simulink model "HarnessModel_MotorDriveUnit"  (R2026a)
settings: Solver=daessc  StopTime=10
PreLoadFcn:
  | MDU_HarnessInputs.AxleSpeedSwitch = table( ...
  |   simscape.Value([0 1], "s"), ...
  |   [0 0], ...
  |   VariableNames=["Time" "StepValues"]);
  | 
  | MDU_HarnessInputs.AxleSpeed = table( ...
  |   simscape.Value([0 1 2], "s"), ...
  |   simscape.Value([0 0 0], "rpm"), ...
  |   VariableNames=["Time" "Data"]);
  | 
  | MDU_HarnessInputs.AxleTorque = table( ...
  |   simscape.Value([0 1 2], "s"), ...
  |   simscape.Value([0 0 0], "N*m"), ...
  |   VariableNames=["Time" "Data"]);
  | 
  | MDU_HarnessInputs.MotorTorqueCommand = table( ...
  |   simscape.Value([0 1 2], "s"), ...
  |   simscape.Value([0 0 0], "N*m"), ...
  |   VariableNames=["Time" "Data"]);
  | 
  | MDU_HarnessInputs.MotorHeatFlow = table( ...
  |   simscape.Value([0 1 2], "s"), ...
  |   simscape.Value([0 0 0], "W"), ...
  |   VariableNames=["Time" "Data"]);
  | 
  | setupHarness_MotorDriveUnit
undefined symbols (not defined in the file or in its folder): BatteryHV, initial, MechanicalLoad, Minus, Plus
libraries: fl_lib x22, nesl_utility x10, sdl_lib x1
settings Model: Creator=isaacito  LastModifiedBy=ythvg
settings SimscapeCC: SimscapeNominalValues="[{\"value\":\"1\",\"unit\":\"A\"},{\"value\":\"1\",\"unit\":\"bar\"},{\"value\":\"1\",\"unit\":\"cm^2\"},{\"value\":\"1\",\"unit\":\"cm^3/s\"},{\"value\":\"1\",\"unit\":\"kJ/kg\"},{\"value\":\"1\",\"unit\":\"kW\"},{\"value\":\"1\",\"unit\":\"l\"},{\"value\":\"1\",\"unit\":\"N\"},{\"value\":\"1\",\"unit\":\"N*m\"},{\"value\":\"1\",\"unit\":\"V\"}]"  SimscapeLogSimulationStatistics=on  SimscapeLogLimitData=off  SimscapeLogDataHistory=5000.0

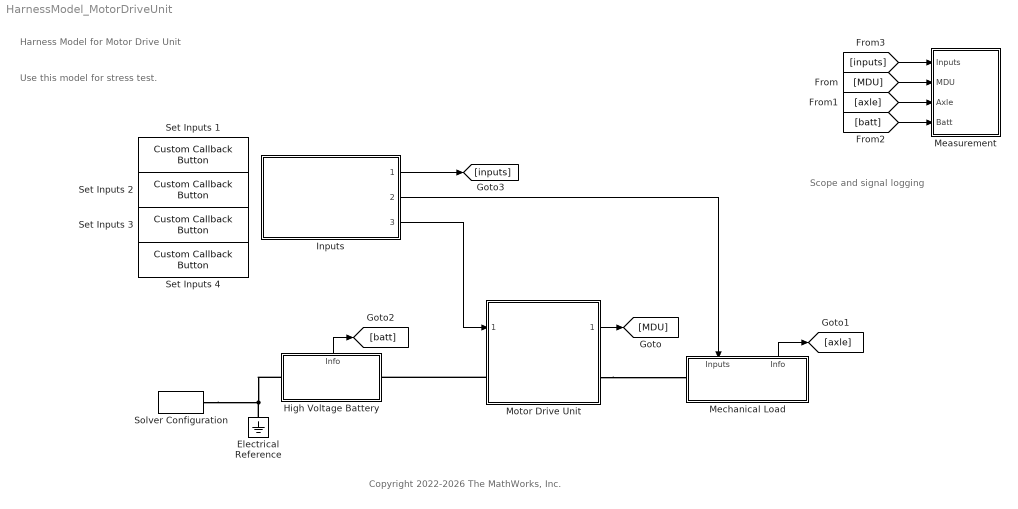
== system HarnessModel_MotorDriveUnit ==
  note: Harness Model for Motor Drive Unit
  note: Copyright 2022-2026 The MathWorks, Inc.
  note: Use this model for stress test.
  note: Scope and signal logging
  Electrical Reference : fl_lib/Electrical/Electrical Elements/Electrical Reference
  High Voltage Battery : Subsystem
      settings: PortSchema="{\"entries\":[{\"content\":{\"sides\":[{\"content\":{\"connectorIds\":[\"LConn1\"]},\"type\":\"ConnectorPlacement.EquallySpacedRectSide\",\"uuid\":\"8acd7e9a-bb08-4de6-aa14-0989ebba81b9\"},{\"content\":{\"connectorIds\":[\"RConn1\"],\"side\":\"RIGHT\"},\"type\":\"ConnectorPlacement.EquallySpacedRectSide\",\"uuid\":\"f80e1afc-966f-4d6b-84f9-f0b60dd6f20c\"},{\"content\":{\"connectorIds\":[\"Out1\"],\"side\":\"TOP\"},\"type\":\"ConnectorPlacement.EquallySpacedRectSide\",\"uuid\":\"52ccb2b1-bd5e-4dcb-b9b6-0ef03b912c33\"}]},\"type\":\"ConnectorPlacement.EquallySpacedConnector\",\"uuid\":\"b55f48a4-f283-4a77-8513-99b31abb285a\"}],\"packageUris\":[\"http://schema.mathworks.com/mf0/Connector/R2020b\"],\"version\":\"1.0\"}"
  Inputs : Subsystem  ReferencedSubsystem=Inputs_MotorDriveUnit_LookupTable_refsub
      settings: OpenFcn="open_system(gcb, \"force\")"
  Measurement : Subsystem
  Mechanical Load : Subsystem
      settings: PortSchema="{\"entries\":[{\"content\":{\"sides\":[{\"content\":{\"connectorIds\":[\"LConn1\"]},\"type\":\"ConnectorPlacement.EquallySpacedRectSide\",\"uuid\":\"18221845-08ef-4cf2-b090-320221152030\"},{\"content\":{\"connectorIds\":[],\"side\":\"RIGHT\"},\"type\":\"ConnectorPlacement.EquallySpacedRectSide\",\"uuid\":\"d5b0548b-74c8-455a-9783-7dc299f3571f\"},{\"content\":{\"connectorIds\":[\"In1\",\"Out1\"],\"side\":\"TOP\"},\"type\":\"ConnectorPlacement.EquallySpacedRectSide\",\"uuid\":\"542d8e55-6d7f-4c9a-9fdc-66897ed9f466\"}]},\"type\":\"ConnectorPlacement.EquallySpacedConnector\",\"uuid\":\"3cd4c536-0337-4305-a842-969bfb1fefe3\"}],\"packageUris\":[\"http://schema.mathworks.com/mf0/Connector/R2020b\"],\"version\":\"1.0\"}"
  Motor Drive Unit : Subsystem  ReferencedSubsystem=MotorDriveUnit_Basic_refsub
      settings: OpenFcn=|
      | % Look under mask:
      | open_system(gcb, "force")
  Set Inputs 1 : CustomCallbackButton  Configuration="{\"components\":[{\"name\":\"BackgroundImageComponent\",\"settings\":{\"image\":{\"size\":[0,0],\"src\":\"default\",\"srcOrientation\":\"Right\"},\"position\":[0,0,1,1]}},{\"name\":\"ButtonStateComponent\",\"settings\":{\"buttonType\":\"momentary\",\"clickFcn\":\"disp(\\\"Loading inputs: <a href=\\\"\\\"matlab:edit('LoadInputs_MotorDriveUnit_zero')\\\"\\\">LoadInputs_MotorDriveUnit_zero<\\/a>\\\")\\nLoadInputs_MotorDriveUnit_zero\\n\\nset_param(bdroot, StopTime=\\\"10\\\")\\nset_param(gcs + \\\"\\/Inputs\\\", ReferencedSubsystem = \\\"Inputs_MotorDriveUnit_LookupTable_refsub\\\")\\n\",\"onValue\":1,\"position\":[0,0,1,1],\"pressDelay\":\"500\",\"pressFcn\":\"\",\"repeatInterval\":\"0\",\"states\":[{\"horizontalAlignment\":\"center\",\"image\":{\"position\":[0,0,1,1],\"size\":[1,1],\"src\":\"default\",\"srcOrientation\":\"Right\"},\"label\":{\"color\":[0.01176470588,0.01176470588,0.01176470588,1],\"icon\":{\"size\":[0,0],\"src\":\"default\",\"srcOrientation\":\"Right\"},\"iconOffset\":0,\"iconPlacement\":\"left\",\"opacity\":1,\"show\":true,\"text\":{\"content\":\"Constant\",\"font\":\"Helvetica\"}},\"labelOffset\":[0,0],\"verticalAlignment\":\"middle\"},{\"horizontalAlignment\":\"center\",\"image\":{\"position\":[0,0,1,1],\"size\":[1,1],\"src\":\"default\",\"srcOrientation\":\"Right\"},\"label\":{\"color\":[0.01176470588,0.01176470588,0.01176470588,1],\"icon\":{\"size\":[0,0],\"src\":\"default\",\"srcOrientation\":\"Right\"},\"iconOffset\":0,\"iconPlacement\":\"left\",\"opacity\":1,\"show\":true,\"text\":{\"content\":\"Constant\",\"font\":\"Helvetica\"}},\"labelOffset\":[0,0],\"verticalAlignment\":\"middle\"},{\"horizontalAlignment\":\"center\",\"image\":{\"position\":[0,0,1,1],\"size\":[1,1],\"src\":\"default\",\"srcOrientation\":\"Right\"},\"label\":{\"color\":[0.01176470588,0.01176470588,0.01176470588,1],\"icon\":{\"size\":[0,0],\"src\":\"default\",\"srcOrientation\":\"Right\"},\"iconOffset\":0,\"iconPlacement\":\"left\",\"opacity\":1,\"show\":true,\"text\":{\"content\":\"Constant\",\"font\":\"Helvetica\"}},\"labelOffset\":[0,0],\"verticalAlignment\":\"middle\"},{\"horizontalAlignment\":\"center\",\"image\":{\"position\":[0,0,1,1],\"size\":[1,1],\"src\":\"default\",\"srcOrientation\":\"Right\"},\"label\":{\"color\":[0.01176470588,0.01176470588,0.01176470588,1],\"icon\":{\"size\":[0,0],\"src\":\"default\",\"srcOrientation\":\"Right\"},\"iconOffset\":0,\"iconPlacement\":\"left\",\"opacity\":1,\"show\":true,\"text\":{\"content\":\"Constant\",\"font\":\"Helvetica\"}},\"labelOffset\":[0,0],\"verticalAlignment\":\"middle\"}]}},{\"name\":\"ForegroundImageComponent\",\"settings\":{\"image\":{\"size\":[0,0],\"src\":\"default\",\"srcOrientation\":\"Right\"},\"isForeground\":1,\"position\":[0,0,1,1]}}],\"derived\":{\"blockParameters\":{\"AutoActivate\":true,\"ButtonText\":\"Constant\",\"ButtonType\":\"Momentary\",\"ClickFcn\":\"disp(\\\"Loading inputs: <a href=\\\"\\\"matlab:edit('LoadInputs_MotorDriveUnit_zero')\\\"\\\">LoadInputs_MotorDriveUnit_zero<\\/a>\\\")\\nLoadInputs_MotorDriveUnit_zero\\n\\nset_param(bdroot, StopTime=\\\"10\\\")\\nset_param(gcs + \\\"\\/Inputs\\\", ReferencedSubsystem = \\\"Inputs_MotorDriveUnit_LookupTable_refsub\\\")\\n\",\"OnValue\":1,\"PressDelay\":\"500\",\"PressFcn\":\"\",\"RepeatInterval\":\"0\",\"fixedAspectRatio\":\"on\"}},\"settings\":{\"BindingType\":\"standalone\",\"autoActivate\":true,\"backgroundColor\":[244,244,244,1],\"backgroundOffset\":0.2,\"backgroundOpacity\":1,\"fixedAspectRatio\":\"on\",\"foregroundColor\":[0.01176470588,0.01176470588,0.01176470588,1],\"migratedFromLegacy\":true,\"useBackgroundColor\":true,\"variant\":\"callback\",\"version\":\"R2025a\"},\"type\":\"Button\"}"  CustomBackgroundColor="{\"color\":[0.9568627451,0.9568627451,0.9568627451],\"show\":true}"
  Set Inputs 2 : CustomCallbackButton  Configuration="{\"components\":[{\"name\":\"BackgroundImageComponent\",\"settings\":{\"image\":{\"size\":[0,0],\"src\":\"default\",\"srcOrientation\":\"Right\"},\"position\":[0,0,1,1]}},{\"name\":\"ButtonStateComponent\",\"settings\":{\"buttonType\":\"momentary\",\"clickFcn\":\"disp(\\\"Loading inputs: <a href=\\\"\\\"matlab:edit('LoadInputs_MotorDriveUnit_Drive')\\\"\\\">LoadInputs_MotorDriveUnit_Drive<\\/a>\\\")\\nLoadInputs_MotorDriveUnit_Drive\\n\\nset_param(bdroot, StopTime=\\\"300\\\")\\nset_param(gcs + \\\"\\/Inputs\\\", ReferencedSubsystem = \\\"Inputs_MotorDriveUnit_LookupTable_refsub\\\")\\n\",\"onValue\":1,\"position\":[0,0,1,1],\"pressDelay\":\"500\",\"pressFcn\":\"\",\"repeatInterval\":\"0\",\"states\":[{\"horizontalAlignment\":\"center\",\"image\":{\"position\":[0,0,1,1],\"size\":[1,1],\"src\":\"default\",\"srcOrientation\":\"Right\"},\"label\":{\"color\":[0.01176470588,0.01176470588,0.01176470588,1],\"icon\":{\"size\":[0,0],\"src\":\"default\",\"srcOrientation\":\"Right\"},\"iconOffset\":0,\"iconPlacement\":\"left\",\"opacity\":1,\"show\":true,\"text\":{\"content\":\"Drive\",\"font\":\"Helvetica\"}},\"labelOffset\":[0,0],\"verticalAlignment\":\"middle\"},{\"horizontalAlignment\":\"center\",\"image\":{\"position\":[0,0,1,1],\"size\":[1,1],\"src\":\"default\",\"srcOrientation\":\"Right\"},\"label\":{\"color\":[0.01176470588,0.01176470588,0.01176470588,1],\"icon\":{\"size\":[0,0],\"src\":\"default\",\"srcOrientation\":\"Right\"},\"iconOffset\":0,\"iconPlacement\":\"left\",\"opacity\":1,\"show\":true,\"text\":{\"content\":\"Drive\",\"font\":\"Helvetica\"}},\"labelOffset\":[0,0],\"verticalAlignment\":\"middle\"},{\"horizontalAlignment\":\"center\",\"image\":{\"position\":[0,0,1,1],\"size\":[1,1],\"src\":\"default\",\"srcOrientation\":\"Right\"},\"label\":{\"color\":[0.01176470588,0.01176470588,0.01176470588,1],\"icon\":{\"size\":[0,0],\"src\":\"default\",\"srcOrientation\":\"Right\"},\"iconOffset\":0,\"iconPlacement\":\"left\",\"opacity\":1,\"show\":true,\"text\":{\"content\":\"Drive\",\"font\":\"Helvetica\"}},\"labelOffset\":[0,0],\"verticalAlignment\":\"middle\"},{\"horizontalAlignment\":\"center\",\"image\":{\"position\":[0,0,1,1],\"size\":[1,1],\"src\":\"default\",\"srcOrientation\":\"Right\"},\"label\":{\"color\":[0.01176470588,0.01176470588,0.01176470588,1],\"icon\":{\"size\":[0,0],\"src\":\"default\",\"srcOrientation\":\"Right\"},\"iconOffset\":0,\"iconPlacement\":\"left\",\"opacity\":1,\"show\":true,\"text\":{\"content\":\"Drive\",\"font\":\"Helvetica\"}},\"labelOffset\":[0,0],\"verticalAlignment\":\"middle\"}]}},{\"name\":\"ForegroundImageComponent\",\"settings\":{\"image\":{\"size\":[0,0],\"src\":\"default\",\"srcOrientation\":\"Right\"},\"isForeground\":1,\"position\":[0,0,1,1]}}],\"derived\":{\"blockParameters\":{\"AutoActivate\":true,\"ButtonText\":\"Drive\",\"ButtonType\":\"Momentary\",\"ClickFcn\":\"disp(\\\"Loading inputs: <a href=\\\"\\\"matlab:edit('LoadInputs_MotorDriveUnit_Drive')\\\"\\\">LoadInputs_MotorDriveUnit_Drive<\\/a>\\\")\\nLoadInputs_MotorDriveUnit_Drive\\n\\nset_param(bdroot, StopTime=\\\"300\\\")\\nset_param(gcs + \\\"\\/Inputs\\\", ReferencedSubsystem = \\\"Inputs_MotorDriveUnit_LookupTable_refsub\\\")\\n\",\"OnValue\":1,\"PressDelay\":\"500\",\"PressFcn\":\"\",\"RepeatInterval\":\"0\",\"fixedAspectRatio\":\"on\"}},\"settings\":{\"BindingType\":\"standalone\",\"autoActivate\":true,\"backgroundColor\":[244,244,244,1],\"backgroundOffset\":0.2,\"backgroundOpacity\":1,\"fixedAspectRatio\":\"on\",\"foregroundColor\":[0.01176470588,0.01176470588,0.01176470588,1],\"migratedFromLegacy\":true,\"useBackgroundColor\":true,\"variant\":\"callback\",\"version\":\"R2025a\"},\"type\":\"Button\"}"  CustomBackgroundColor="{\"color\":[0.9568627451,0.9568627451,0.9568627451],\"show\":true}"
  Set Inputs 3 : CustomCallbackButton  Configuration="{\"components\":[{\"name\":\"BackgroundImageComponent\",\"settings\":{\"image\":{\"size\":[0,0],\"src\":\"default\",\"srcOrientation\":\"Right\"},\"position\":[0,0,1,1]}},{\"name\":\"ButtonStateComponent\",\"settings\":{\"buttonType\":\"momentary\",\"clickFcn\":\"disp(\\\"Loading inputs: <a href=\\\"\\\"matlab:edit('LoadInputs_MotorDriveUnit_Regen')\\\"\\\">LoadInputs_MotorDriveUnit_Regen<\\/a>\\\")\\nLoadInputs_MotorDriveUnit_Regen\\n\\nset_param(bdroot, StopTime=\\\"400\\\")\\nset_param(gcs + \\\"\\/Inputs\\\", ReferencedSubsystem = \\\"Inputs_MotorDriveUnit_LookupTable_refsub\\\")\\n\",\"onValue\":1,\"position\":[0,0,1,1],\"pressDelay\":\"500\",\"pressFcn\":\"\",\"repeatInterval\":\"0\",\"states\":[{\"horizontalAlignment\":\"center\",\"image\":{\"position\":[0,0,1,1],\"size\":[1,1],\"src\":\"default\",\"srcOrientation\":\"Right\"},\"label\":{\"color\":[0.01176470588,0.01176470588,0.01176470588,1],\"icon\":{\"size\":[0,0],\"src\":\"default\",\"srcOrientation\":\"Right\"},\"iconOffset\":0,\"iconPlacement\":\"left\",\"opacity\":1,\"show\":true,\"text\":{\"content\":\"Regen Brake\",\"font\":\"Helvetica\"}},\"labelOffset\":[0,0],\"verticalAlignment\":\"middle\"},{\"horizontalAlignment\":\"center\",\"image\":{\"position\":[0,0,1,1],\"size\":[1,1],\"src\":\"default\",\"srcOrientation\":\"Right\"},\"label\":{\"color\":[0.01176470588,0.01176470588,0.01176470588,1],\"icon\":{\"size\":[0,0],\"src\":\"default\",\"srcOrientation\":\"Right\"},\"iconOffset\":0,\"iconPlacement\":\"left\",\"opacity\":1,\"show\":true,\"text\":{\"content\":\"Regen Brake\",\"font\":\"Helvetica\"}},\"labelOffset\":[0,0],\"verticalAlignment\":\"middle\"},{\"horizontalAlignment\":\"center\",\"image\":{\"position\":[0,0,1,1],\"size\":[1,1],\"src\":\"default\",\"srcOrientation\":\"Right\"},\"label\":{\"color\":[0.01176470588,0.01176470588,0.01176470588,1],\"icon\":{\"size\":[0,0],\"src\":\"default\",\"srcOrientation\":\"Right\"},\"iconOffset\":0,\"iconPlacement\":\"left\",\"opacity\":1,\"show\":true,\"text\":{\"content\":\"Regen Brake\",\"font\":\"Helvetica\"}},\"labelOffset\":[0,0],\"verticalAlignment\":\"middle\"},{\"horizontalAlignment\":\"center\",\"image\":{\"position\":[0,0,1,1],\"size\":[1,1],\"src\":\"default\",\"srcOrientation\":\"Right\"},\"label\":{\"color\":[0.01176470588,0.01176470588,0.01176470588,1],\"icon\":{\"size\":[0,0],\"src\":\"default\",\"srcOrientation\":\"Right\"},\"iconOffset\":0,\"iconPlacement\":\"left\",\"opacity\":1,\"show\":true,\"text\":{\"content\":\"Regen Brake\",\"font\":\"Helvetica\"}},\"labelOffset\":[0,0],\"verticalAlignment\":\"middle\"}]}},{\"name\":\"ForegroundImageComponent\",\"settings\":{\"image\":{\"size\":[0,0],\"src\":\"default\",\"srcOrientation\":\"Right\"},\"isForeground\":1,\"position\":[0,0,1,1]}}],\"derived\":{\"blockParameters\":{\"AutoActivate\":true,\"ButtonText\":\"Regen Brake\",\"ButtonType\":\"Momentary\",\"ClickFcn\":\"disp(\\\"Loading inputs: <a href=\\\"\\\"matlab:edit('LoadInputs_MotorDriveUnit_Regen')\\\"\\\">LoadInputs_MotorDriveUnit_Regen<\\/a>\\\")\\nLoadInputs_MotorDriveUnit_Regen\\n\\nset_param(bdroot, StopTime=\\\"400\\\")\\nset_param(gcs + \\\"\\/Inputs\\\", ReferencedSubsystem = \\\"Inputs_MotorDriveUnit_LookupTable_refsub\\\")\\n\",\"OnValue\":1,\"PressDelay\":\"500\",\"PressFcn\":\"\",\"RepeatInterval\":\"0\",\"fixedAspectRatio\":\"on\"}},\"settings\":{\"BindingType\":\"standalone\",\"autoActivate\":true,\"backgroundColor\":[244,244,244,1],\"backgroundOffset\":0.2,\"backgroundOpacity\":1,\"fixedAspectRatio\":\"on\",\"foregroundColor\":[0.01176470588,0.01176470588,0.01176470588,1],\"migratedFromLegacy\":true,\"useBackgroundColor\":true,\"variant\":\"callback\",\"version\":\"R2025a\"},\"type\":\"Button\"}"  CustomBackgroundColor="{\"color\":[0.9568627451,0.9568627451,0.9568627451],\"show\":true}"
  Set Inputs 4 : CustomCallbackButton  Configuration="{\"components\":[{\"name\":\"BackgroundImageComponent\",\"settings\":{\"image\":{\"size\":[0,0],\"src\":\"default\",\"srcOrientation\":\"Right\"},\"position\":[0,0,1,1]}},{\"name\":\"ButtonStateComponent\",\"settings\":{\"buttonType\":\"momentary\",\"clickFcn\":\"disp(\\\"Loading inputs: <a href=\\\"\\\"matlab:edit('LoadInputs_MotorDriveUnit_Random')\\\"\\\">LoadInputs_MotorDriveUnit_Random<\\/a>\\\")\\nLoadInputs_MotorDriveUnit_Random\\n\\nset_param(bdroot, StopTime=\\\"400\\\")\\nset_param(gcs + \\\"\\/Inputs\\\", ReferencedSubsystem = \\\"Inputs_MotorDriveUnit_LookupTable_refsub\\\")\\n\",\"onValue\":1,\"position\":[0,0,1,1],\"pressDelay\":\"500\",\"pressFcn\":\"\",\"repeatInterval\":\"0\",\"states\":[{\"horizontalAlignment\":\"center\",\"image\":{\"position\":[0,0,1,1],\"size\":[1,1],\"src\":\"default\",\"srcOrientation\":\"Right\"},\"label\":{\"color\":[0.01176470588,0.01176470588,0.01176470588,1],\"icon\":{\"size\":[0,0],\"src\":\"default\",\"srcOrientation\":\"Right\"},\"iconOffset\":0,\"iconPlacement\":\"left\",\"opacity\":1,\"show\":true,\"text\":{\"content\":\"Random\",\"font\":\"Helvetica\"}},\"labelOffset\":[0,0],\"verticalAlignment\":\"middle\"},{\"horizontalAlignment\":\"center\",\"image\":{\"position\":[0,0,1,1],\"size\":[1,1],\"src\":\"default\",\"srcOrientation\":\"Right\"},\"label\":{\"color\":[0.01176470588,0.01176470588,0.01176470588,1],\"icon\":{\"size\":[0,0],\"src\":\"default\",\"srcOrientation\":\"Right\"},\"iconOffset\":0,\"iconPlacement\":\"left\",\"opacity\":1,\"show\":true,\"text\":{\"content\":\"Random\",\"font\":\"Helvetica\"}},\"labelOffset\":[0,0],\"verticalAlignment\":\"middle\"},{\"horizontalAlignment\":\"center\",\"image\":{\"position\":[0,0,1,1],\"size\":[1,1],\"src\":\"default\",\"srcOrientation\":\"Right\"},\"label\":{\"color\":[0.01176470588,0.01176470588,0.01176470588,1],\"icon\":{\"size\":[0,0],\"src\":\"default\",\"srcOrientation\":\"Right\"},\"iconOffset\":0,\"iconPlacement\":\"left\",\"opacity\":1,\"show\":true,\"text\":{\"content\":\"Random\",\"font\":\"Helvetica\"}},\"labelOffset\":[0,0],\"verticalAlignment\":\"middle\"},{\"horizontalAlignment\":\"center\",\"image\":{\"position\":[0,0,1,1],\"size\":[1,1],\"src\":\"default\",\"srcOrientation\":\"Right\"},\"label\":{\"color\":[0.01176470588,0.01176470588,0.01176470588,1],\"icon\":{\"size\":[0,0],\"src\":\"default\",\"srcOrientation\":\"Right\"},\"iconOffset\":0,\"iconPlacement\":\"left\",\"opacity\":1,\"show\":true,\"text\":{\"content\":\"Random\",\"font\":\"Helvetica\"}},\"labelOffset\":[0,0],\"verticalAlignment\":\"middle\"}]}},{\"name\":\"ForegroundImageComponent\",\"settings\":{\"image\":{\"size\":[0,0],\"src\":\"default\",\"srcOrientation\":\"Right\"},\"isForeground\":1,\"position\":[0,0,1,1]}}],\"derived\":{\"blockParameters\":{\"AutoActivate\":true,\"ButtonText\":\"Random\",\"ButtonType\":\"Momentary\",\"ClickFcn\":\"disp(\\\"Loading inputs: <a href=\\\"\\\"matlab:edit('LoadInputs_MotorDriveUnit_Random')\\\"\\\">LoadInputs_MotorDriveUnit_Random<\\/a>\\\")\\nLoadInputs_MotorDriveUnit_Random\\n\\nset_param(bdroot, StopTime=\\\"400\\\")\\nset_param(gcs + \\\"\\/Inputs\\\", ReferencedSubsystem = \\\"Inputs_MotorDriveUnit_LookupTable_refsub\\\")\\n\",\"OnValue\":1,\"PressDelay\":\"500\",\"PressFcn\":\"\",\"RepeatInterval\":\"0\",\"fixedAspectRatio\":\"on\"}},\"settings\":{\"BindingType\":\"standalone\",\"autoActivate\":true,\"backgroundColor\":[244,244,244,1],\"backgroundOffset\":0.2,\"backgroundOpacity\":1,\"fixedAspectRatio\":\"on\",\"foregroundColor\":[0.01176470588,0.01176470588,0.01176470588,1],\"migratedFromLegacy\":true,\"useBackgroundColor\":true,\"variant\":\"callback\",\"version\":\"R2025a\"},\"type\":\"Button\"}"  CustomBackgroundColor="{\"color\":[0.9568627451,0.9568627451,0.9568627451],\"show\":true}"
  Solver Configuration : nesl_utility/Solver Configuration  PhysicalDomain=network_engine_domain  SubClassName=solver  LeftPortType=input  RightPortType=generic  Tones=[]  Harmonics=[]  SimulateNoise=off  Profile=off  UseLocalSampling=off  EnableSwitchedLinearOptims=on  FrequencyDomain=off  UseCCode=off  RelTol=0.001  AbsTol=1e-06  MinStep=1e-09  ToWorkspace=off  RevertToSquareIcSolve=off  NumHomotopyIterations=100  PhasorMode=off  PhasorModeNumHarmonics=1  ConsistencySolver=NEWTON_FTOL  CanonicalOrdering=UNORDERED  OptimizeIntermediates=UNOPTIMIZED  IndexReductionMethod=DerivativeReplacement  DoDC=off  ResidualTolerance=1e-09  ConsistencyTolSource=GLOBAL  ConsistencyAbsTol=0.001  ConsistencyRelTol=0.001  ConsistencyTolFactor=0.001  UseLocalSolver=off  LocalSolverChoice=NE_BACKWARD_EULER_ADVANCER  ResolveIndetEquations=on  FunctionEvalNumThread=1  LocalSolverSampleTime=0.001  DoFixedCost=off  MaxNonlinIter=3  MaxModeIter=2  ComputeImpulses=off  ImpulseIterations=2  LinearAlgebra=auto  LinearAlgebraNumThread=0  EquationFormulation=NE_TIME_EF  DelaysMemoryBudget=1024  AutomaticFiltering=on  FilteringTimeConstant=0.001  PartitionStorageMethod=AS_NEEDED  PartitionMemoryBudget=1024  PartitionMethod=ROBUST  MultibodyUseLocalSolver=off  MultibodyLocalSolverChoice=ODE1  MultibodyLocalSolverSampleTime=0.001
      settings: AttributesFormatString=Local solver %<UseLocalSolver>
  wires:
  Motor Drive Unit/1 -> [MDU]
  [MDU] -> Measurement/2(MDU)
  Inputs/3 -> Motor Drive Unit/1
  [axle] -> Measurement/3(Axle)
  High Voltage Battery/1(Info) -> [batt]
  [batt] -> Measurement/4(Batt)
  Inputs/2 -> Mechanical Load/1(Inputs)
  Mechanical Load/1(Info) -> [axle]
  Inputs/1 -> [inputs]
  [inputs] -> Measurement/1(Inputs)
  connections:
  Motor Drive Unit/LConn1 -- High Voltage Battery/RConn1
  Electrical Reference/LConn1 -- High Voltage Battery/LConn1 -- Solver Configuration/RConn1
  Motor Drive Unit/RConn1 -- Mechanical Load/LConn1

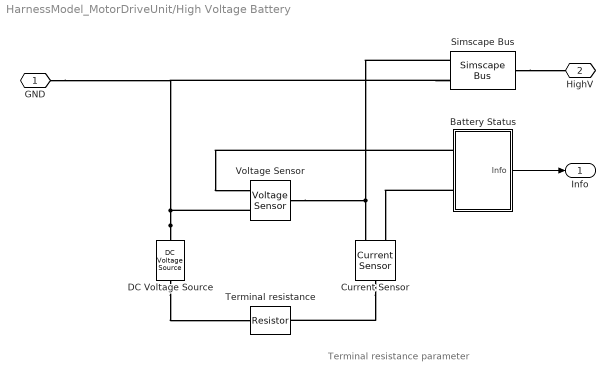
== system HarnessModel_MotorDriveUnit/High Voltage Battery ==
  note: Terminal resistance parameter
  Battery Status : Subsystem
  Current Sensor : fl_lib/Electrical/Electrical Sensors/Current Sensor
  DC Voltage Source : fl_lib/Electrical/Electrical Sources/DC Voltage Source  v0="BatteryHV.NominalVoltage.value(\"V\") V"
  Simscape Bus : SimscapeBus  HierarchyStrings=Plus;Minus  ConnectionType=Bus: Bus_HighVoltage
      settings: AttributesFormatString=%<ConnectionType>
  Terminal resistance : fl_lib/Electrical/Electrical Elements/Resistor  R="BatteryHV.TerminalResistance.value(\"Ohm\") Ohm"  i_specify=off  i_priority=High  i=0 A  i_nominal_specify=off  i_nominal_value=1  i_nominal_unit=A  v_specify=off  v_priority=High  v=0 V  v_nominal_specify=off  v_nominal_value=1  v_nominal_unit=V
  Voltage Sensor : fl_lib/Electrical/Electrical Sensors/Voltage Sensor
  GND : PMIOPort  Side=Left
  HighV : PMIOPort  Port=2  Side=Right
  Info : Outport
  wires:
  Battery Status/1(Info) -> Info/1
  connections:
  DC Voltage Source/RConn1 -- GND/RConn1 -- Simscape Bus/LConn2 -- Voltage Sensor/RConn2
  Simscape Bus/LConn1 -- Voltage Sensor/LConn1 -- Current Sensor/RConn2
  Battery Status/LConn2 -- Current Sensor/RConn1
  Simscape Bus/RConn1 -- HighV/RConn1
  Current Sensor/LConn1 -- Terminal resistance/RConn1
  DC Voltage Source/LConn1 -- Terminal resistance/LConn1
  Battery Status/LConn1 -- Voltage Sensor/RConn1

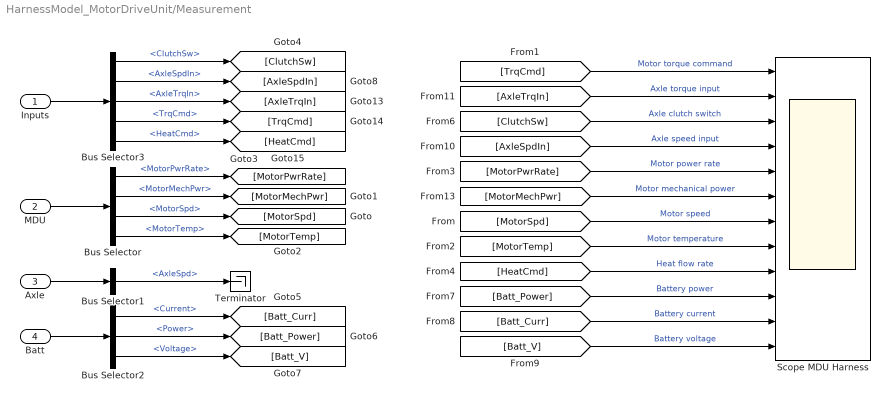
== system HarnessModel_MotorDriveUnit/Measurement ==
  Inputs : Inport
  MDU : Inport  Port=2
  Axle : Inport  Port=3
  Batt : Inport  Port=4
  Bus Selector : BusSelector  OutputSignals=MotorPwrRate,MotorMechPwr,MotorSpd,MotorTemp
  Bus Selector1 : BusSelector  OutputSignals=AxleSpd
  Bus Selector2 : BusSelector  OutputSignals=Current,Power,Voltage
  Bus Selector3 : BusSelector  OutputSignals=signal1.ClutchSw,signal1.AxleSpdIn,signal1.AxleTrqIn,signal2.TrqCmd,signal2.HeatCmd
  Scope MDU Harness : Scope  NumInputPorts=12
      settings: ActiveDisplayYMinimum=-1  ActiveDisplayYMaximum=1
  Terminator : Terminator
  wires:
  MDU/1 -> Bus Selector/1
  Bus Selector/3 -> [MotorSpd]  "<MotorSpd>"
  Bus Selector/4 -> [MotorTemp]  "<MotorTemp>"
  Axle/1 -> Bus Selector1/1
  Bus Selector2/3 -> [Batt_V]  "<Voltage>"
  Bus Selector2/2 -> [Batt_Power]  "<Power>"
  Bus Selector2/1 -> [Batt_Curr]  "<Current>"
  Batt/1 -> Bus Selector2/1
  Bus Selector1/1 -> Terminator/1  "<AxleSpd>"
  Bus Selector/1 -> [MotorPwrRate]  "<MotorPwrRate>"
  Inputs/1 -> Bus Selector3/1
  Bus Selector3/1 -> [ClutchSw]  "<ClutchSw>"
  Bus Selector3/2 -> [AxleSpdIn]  "<AxleSpdIn>"
  Bus Selector3/3 -> [AxleTrqIn]  "<AxleTrqIn>"
  Bus Selector3/4 -> [TrqCmd]  "<TrqCmd>"
  Bus Selector3/5 -> [HeatCmd]  "<HeatCmd>"
  Bus Selector/2 -> [MotorMechPwr]  "<MotorMechPwr>"
  [MotorPwrRate] -> Scope MDU Harness/5  "Motor power rate"
  [TrqCmd] -> Scope MDU Harness/1  "Motor torque command"
  [MotorMechPwr] -> Scope MDU Harness/6  "Motor mechanical power"
  [MotorSpd] -> Scope MDU Harness/7  "Motor speed"
  [MotorTemp] -> Scope MDU Harness/8  "Motor temperature"
  [HeatCmd] -> Scope MDU Harness/9  "Heat flow rate"
  [Batt_Power] -> Scope MDU Harness/10  "Battery power"
  [Batt_Curr] -> Scope MDU Harness/11  "Battery current"
  [Batt_V] -> Scope MDU Harness/12  "Battery voltage"
  [AxleTrqIn] -> Scope MDU Harness/2  "Axle torque input"
  [ClutchSw] -> Scope MDU Harness/3  "Axle clutch switch"
  [AxleSpdIn] -> Scope MDU Harness/4  "Axle speed input"

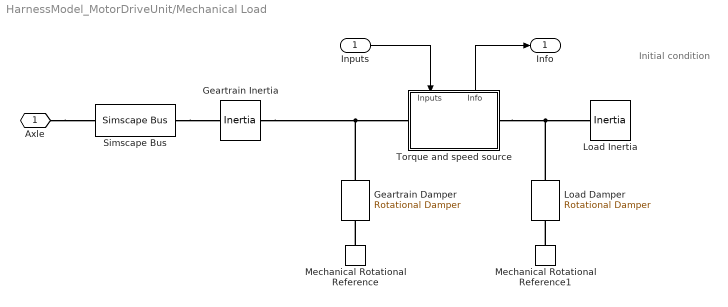
== system HarnessModel_MotorDriveUnit/Mechanical Load ==
  note: Initial condition
  Inputs : Inport
  Geartrain Damper : fl_lib/Mechanical/Rotational Elements/Rotational Damper  D=0.001 m*N/rpm  w_specify=off  w_priority=None  w=0 rad/s  w_nominal_specify=off  w_nominal_value=1  w_nominal_unit=rad/s  t_specify=off  t_priority=None  t=0 N*m  t_nominal_specify=off  t_nominal_value=1  t_nominal_unit=N*m
      settings: AttributesFormatString=|
      | %<D>
      | %<D_unit>
  Geartrain Inertia : fl_lib/Mechanical/Rotational Elements/Inertia  inertia=1.35 kg*m^2  num_ports=foundation.enum.numPorts2.two  w_specify=on  w_priority=None  w=0 rpm  w_nominal_specify=off  w_nominal_value=1  w_nominal_unit=rad/s  t_specify=off  t_priority=None  t=0 N*m  t_nominal_specify=off  t_nominal_value=1  t_nominal_unit=N*m
      settings: AttributesFormatString=|
      | %<inertia> %<inertia_unit>
      | Priority: %<w_priority>
  Load Damper : fl_lib/Mechanical/Rotational Elements/Rotational Damper  D=0.03 N*m/rpm  w_specify=off  w_priority=None  w=0 rad/s  w_nominal_specify=off  w_nominal_value=1  w_nominal_unit=rad/s  t_specify=off  t_priority=None  t=0 N*m  t_nominal_specify=off  t_nominal_value=1  t_nominal_unit=N*m
      settings: AttributesFormatString=|
      | %<D>
      | %<D_unit>
  Load Inertia : fl_lib/Mechanical/Rotational Elements/Inertia  inertia="MechanicalLoad.Inertia.value(\"kg*m^2\") kg*m^2"  num_ports=foundation.enum.numPorts2.one  w_specify=on  w_priority=High  w="initial.LoadInertia_AngularSpeed.value(\"rpm\") rpm"  w_nominal_specify=off  w_nominal_value=1  w_nominal_unit=rad/s  t_specify=off  t_priority=None  t=0 N*m  t_nominal_specify=off  t_nominal_value=1  t_nominal_unit=N*m
      settings: AttributesFormatString=Priority: %<w_priority>
  Mechanical Rotational Reference : fl_lib/Mechanical/Rotational Elements/Mechanical Rotational Reference
  Mechanical Rotational Reference1 : fl_lib/Mechanical/Rotational Elements/Mechanical Rotational Reference
  Simscape Bus : SimscapeBus  HierarchyStrings=AngSpd  ConnectionType=Bus: Bus_Rotational
  Torque and speed source : Subsystem
      settings: PortSchema="{\"entries\":[{\"content\":{\"sides\":[{\"content\":{\"connectorIds\":[\"LConn1\"]},\"type\":\"ConnectorPlacement.EquallySpacedRectSide\",\"uuid\":\"92a06674-aaa2-495f-b380-fd1e5a218eb3\"},{\"content\":{\"connectorIds\":[\"RConn1\"],\"side\":\"RIGHT\"},\"type\":\"ConnectorPlacement.EquallySpacedRectSide\",\"uuid\":\"3e9807eb-b215-4ab1-ac02-6574a58f93c0\"},{\"content\":{\"connectorIds\":[\"In1\",\"Out1\"],\"side\":\"TOP\"},\"type\":\"ConnectorPlacement.EquallySpacedRectSide\",\"uuid\":\"937668c8-63b6-43a7-85c7-81bf7d359316\"}]},\"type\":\"ConnectorPlacement.EquallySpacedConnector\",\"uuid\":\"ba9b6e46-9639-4838-8d50-8636a64d3a24\"}],\"packageUris\":[\"http://schema.mathworks.com/mf0/Connector/R2020b\"],\"version\":\"1.0\"}"
  Axle : PMIOPort  Side=Left
  Info : Outport
  wires:
  Torque and speed source/1(Info) -> Info/1
  Inputs/1 -> Torque and speed source/1(Inputs)
  connections:
  Mechanical Rotational Reference/LConn1 -- Geartrain Damper/RConn1
  Mechanical Rotational Reference1/LConn1 -- Load Damper/RConn1
  Simscape Bus/LConn1 -- Geartrain Inertia/RConn1
  Axle/RConn1 -- Simscape Bus/RConn1
  Torque and speed source/RConn1 -- Load Damper/LConn1 -- Load Inertia/LConn1
  Geartrain Inertia/LConn1 -- Geartrain Damper/LConn1 -- Torque and speed source/LConn1

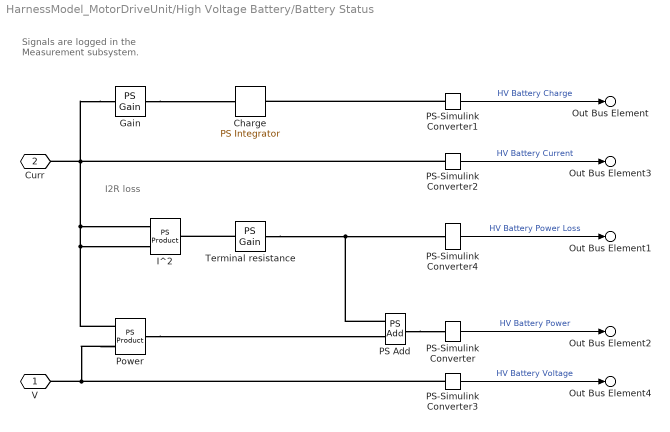
== system HarnessModel_MotorDriveUnit/High Voltage Battery/Battery Status ==
  note: I2R loss
  note: Signals are logged in
      | the Measurement subsystem.
  Charge : fl_lib/Physical Signals/Linear Operators/PS Integrator  reset_method=foundation.enum.IntegratorResetSpec.None  initial_condition_spec=foundation.enum.IntegratorICSpec.Internal  saturation_spec=foundation.enum.IntegratorSaturationSpec.None  saturation_source_spec=foundation.enum.IntegratorSaturationSourceSpec.Internal  x0=0 A*hr  xu=inf s  xl=-inf s
      settings: AttributesFormatString=%<x0> [%<x0_unit>]
  Gain : fl_lib/Physical Signals/Functions/PS Gain  gain=-1
      settings: AttributesFormatString=%<gain>
  I^2 : fl_lib/Physical Signals/Functions/PS Product
  PS Add : fl_lib/Physical Signals/Functions/PS Add
  PS-Simulink Converter : nesl_utility/PS-Simulink Converter  PhysicalDomain=network_engine_domain  SubClassName=ps_output  LeftPortType=input  RightPortType=output  PseudoPeriodic=off  Frequencies=[]  VectorFormat=1-D array  Unit=kW  AffineConversion=off
  PS-Simulink Converter1 : nesl_utility/PS-Simulink Converter  PhysicalDomain=network_engine_domain  SubClassName=ps_output  LeftPortType=input  RightPortType=output  PseudoPeriodic=off  Frequencies=[]  VectorFormat=1-D array  Unit=A*hr  AffineConversion=off
  PS-Simulink Converter2 : nesl_utility/PS-Simulink Converter  PhysicalDomain=network_engine_domain  SubClassName=ps_output  LeftPortType=input  RightPortType=output  PseudoPeriodic=off  Frequencies=[]  VectorFormat=1-D array  Unit=A  AffineConversion=off
  PS-Simulink Converter3 : nesl_utility/PS-Simulink Converter  PhysicalDomain=network_engine_domain  SubClassName=ps_output  LeftPortType=input  RightPortType=output  PseudoPeriodic=off  Frequencies=[]  VectorFormat=1-D array  Unit=V  AffineConversion=off
  PS-Simulink Converter4 : nesl_utility/PS-Simulink Converter  PhysicalDomain=network_engine_domain  SubClassName=ps_output  LeftPortType=input  RightPortType=output  PseudoPeriodic=off  Frequencies=[]  VectorFormat=1-D array  Unit=W  AffineConversion=off
  Power : fl_lib/Physical Signals/Functions/PS Product
  Terminal resistance : fl_lib/Physical Signals/Functions/PS Gain  gain="BatteryHV.TerminalResistance.value(\"Ohm\") Ohm"
  V : PMIOPort  Side=Left
  Curr : PMIOPort  Port=2  Side=Left
  Out Bus Element : Outport  PortName=Info  Element=Charge
      settings: AttributesFormatString=%<Unit>
  Out Bus Element3 : Outport  PortName=Info  Element=Current
      settings: AttributesFormatString=%<Unit>
  Out Bus Element1 : Outport  PortName=Info  Element=PowerLoss
      settings: AttributesFormatString=%<Unit>
  Out Bus Element2 : Outport  PortName=Info  Element=Power
      settings: AttributesFormatString=%<Unit>
  Out Bus Element4 : Outport  PortName=Info  Element=Voltage
      settings: AttributesFormatString=%<Unit>
  wires:
  PS-Simulink Converter3/1 -> Out Bus Element4/1  "HV Battery Voltage"
  PS-Simulink Converter2/1 -> Out Bus Element3/1  "HV Battery Current"
  PS-Simulink Converter4/1 -> Out Bus Element1/1  "HV Battery Power Loss"
  PS-Simulink Converter1/1 -> Out Bus Element/1  "HV Battery Charge"
  PS-Simulink Converter/1 -> Out Bus Element2/1  "HV Battery Power"
  connections:
  Power/RConn1 -- PS Add/LConn2
  PS Add/RConn1 -- PS-Simulink Converter/LConn1
  Terminal resistance/LConn1 -- I^2/RConn1
  PS-Simulink Converter1/LConn1 -- Charge/RConn1
  Gain/RConn1 -- Charge/LConn1
  PS Add/LConn1 -- PS-Simulink Converter4/LConn1 -- Terminal resistance/RConn1
  Power/LConn1 -- V/RConn1 -- PS-Simulink Converter3/LConn1
  Gain/LConn1 -- PS-Simulink Converter2/LConn1 -- Curr/RConn1 -- I^2/LConn1 -- Power/LConn2 -- I^2/LConn2

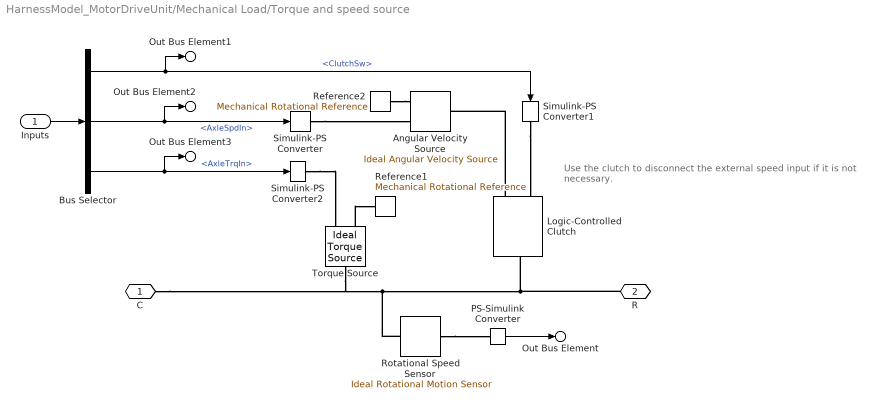
== system HarnessModel_MotorDriveUnit/Mechanical Load/Torque and speed source ==
  note: Use the clutch to disconnect the external speed input if it is not necessary.
  Inputs : Inport
  Angular Velocity Source : fl_lib/Mechanical/Mechanical Sources/Ideal Angular Velocity Source
  Bus Selector : BusSelector  OutputSignals=ClutchSw,AxleSpdIn,AxleTrqIn
  Logic-Controlled Clutch : sdl_lib/Clutches/Logic-Controlled Clutch  transition_model=sdl.enum.transitionModel.instant  transition_time_constant=0.1 s  t_friction=5000 N*m  t_locked=5000 N*m  w_tol=0.1 rpm  initial_state_locked=sdl.enum.initial_lock.unlocked
  PS-Simulink Converter : nesl_utility/PS-Simulink Converter  PhysicalDomain=network_engine_domain  SubClassName=ps_output  LeftPortType=input  RightPortType=output  PseudoPeriodic=off  Frequencies=[]  VectorFormat=inherit  Unit=rpm  AffineConversion=off
  Reference1 : fl_lib/Mechanical/Rotational Elements/Mechanical Rotational Reference
  Reference2 : fl_lib/Mechanical/Rotational Elements/Mechanical Rotational Reference
  Rotational Speed Sensor : fl_lib/Mechanical/Mechanical Sensors/Ideal Rotational Motion Sensor  reference=foundation.enum.MeasurementReference.absolute  acceleration_port=false  velocity_port=true  position_port=false  wrap_angle=simscape.enum.onoff.off  offset=0 rad
  Simulink-PS Converter : nesl_utility/Simulink-PS Converter  PhysicalDomain=network_engine_domain  SubClassName=ps_input  LeftPortType=input  RightPortType=output  PseudoPeriodic=off  Frequencies=[]  NoiseDistribution=none  NoiseParameters=[]  Unit=rpm  AffineConversion=off  FilteringAndDerivatives=filter  SimscapeFilterOrder=1  InputFilterTimeConstant=0.001  UdotUserProvided=1
  Simulink-PS Converter2 : nesl_utility/Simulink-PS Converter  PhysicalDomain=network_engine_domain  SubClassName=ps_input  LeftPortType=input  RightPortType=output  PseudoPeriodic=off  Frequencies=[]  NoiseDistribution=none  NoiseParameters=[]  Unit=N*m  AffineConversion=off  FilteringAndDerivatives=filter  SimscapeFilterOrder=1  InputFilterTimeConstant=0.001  UdotUserProvided=1
  Simulink-PS Converter1 : nesl_utility/Simulink-PS Converter  PhysicalDomain=network_engine_domain  SubClassName=ps_input  LeftPortType=input  RightPortType=output  PseudoPeriodic=off  Frequencies=[]  NoiseDistribution=none  NoiseParameters=[]  Unit=1  AffineConversion=off  FilteringAndDerivatives=provide  SimscapeFilterOrder=1  InputFilterTimeConstant=0.001  UdotUserProvided=0
      settings: AttributesFormatString=|
      | %<Unit>
      | Derivative: %<FilteringAndDerivatives>
  Torque Source : fl_lib/Mechanical/Mechanical Sources/Ideal Torque Source
  C : PMIOPort  Side=Left
  R : PMIOPort  Port=2  Side=Right
  Out Bus Element : Outport  PortName=Info  Element=AxleSpd
  Out Bus Element1 : Outport  PortName=Info  Element=AxleClutchSw
  Out Bus Element2 : Outport  PortName=Info  Element=AxleSpdIn
  Out Bus Element3 : Outport  PortName=Info  Element=AxleTrqIn
  wires:
  Inputs/1 -> Bus Selector/1
  Bus Selector/1 -> Out Bus Element1/1, Simulink-PS Converter1/1  "<ClutchSw>"
  Bus Selector/2 -> Simulink-PS Converter/1, Out Bus Element2/1  "<AxleSpdIn>"
  Bus Selector/3 -> Out Bus Element3/1, Simulink-PS Converter2/1  "<AxleTrqIn>"
  PS-Simulink Converter/1 -> Out Bus Element/1
  connections:
  Simulink-PS Converter/RConn1 -- Angular Velocity Source/RConn1
  Reference2/LConn1 -- Angular Velocity Source/RConn2
  Logic-Controlled Clutch/LConn2 -- Angular Velocity Source/LConn1
  Simulink-PS Converter1/RConn1 -- Logic-Controlled Clutch/LConn1
  Rotational Speed Sensor/LConn1 -- C/RConn1 -- Torque Source/LConn1 -- R/RConn1 -- Logic-Controlled Clutch/RConn1
  Rotational Speed Sensor/RConn1 -- PS-Simulink Converter/LConn1
  Simulink-PS Converter2/RConn1 -- Torque Source/RConn1
  Torque Source/RConn2 -- Reference1/LConn1
